simulink model "Parallel_RLC"  (R2025b)
settings: Solver=VariableStepAuto  StartTime=0.0  StopTime=0.03  RelTol=1e-7
libraries: fl_lib x8, nesl_utility x4, ee_lib x1
settings Model: Creator=franc  LastModifiedBy=franc

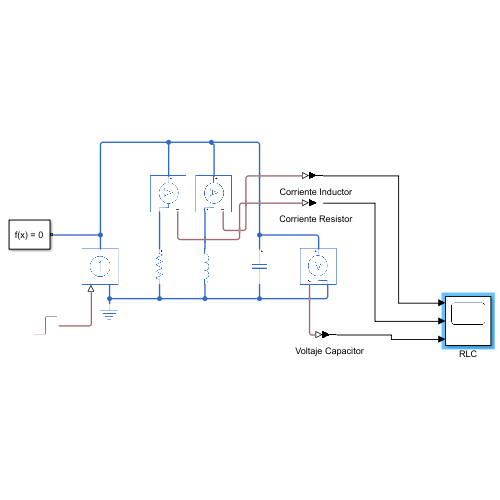
[thumbnail: Simulink's stored preview of the top-level diagram]
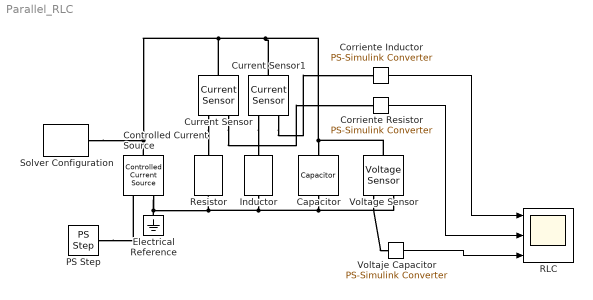
== system Parallel_RLC ==
  Capacitor : fl_lib/Electrical/Electrical Elements/Capacitor  c=2.53e-3 F  r=1e-6 Ohm  g=0 1/Ohm  i_specify=off  i_priority=None  i=0 A  i_nominal_specify=off  i_nominal_value=1  i_nominal_unit=A  v_specify=off  v_priority=None  v=0 V  v_nominal_specify=off  v_nominal_value=1  v_nominal_unit=V  vc_specify=off  vc_priority=High  vc=0 V  vc_nominal_specify=off  vc_nominal_value=1  vc_nominal_unit=V
  Controlled Current Source : fl_lib/Electrical/Electrical Sources/Controlled Current Source
  Corriente Inductor : nesl_utility/PS-Simulink Converter  PhysicalDomain=network_engine_domain  SubClassName=ps_output  LeftPortType=input  RightPortType=output  PseudoPeriodic=off  Frequencies=[]  VectorFormat=inherit  Unit=inherit  AffineConversion=off
  Corriente Resistor : nesl_utility/PS-Simulink Converter  PhysicalDomain=network_engine_domain  SubClassName=ps_output  LeftPortType=input  RightPortType=output  PseudoPeriodic=off  Frequencies=[]  VectorFormat=inherit  Unit=inherit  AffineConversion=off
  Current Sensor : fl_lib/Electrical/Electrical Sensors/Current Sensor
  Current Sensor1 : fl_lib/Electrical/Electrical Sensors/Current Sensor
  Electrical Reference : fl_lib/Electrical/Electrical Elements/Electrical Reference
  Inductor : ee_lib/Passive/Inductor  l=1e-3 H  enable_L_tol=ee.enum.toleranceApplication.none  L_tol=20  tol_distribution=ee.enum.toleranceDistribution.uniform  nSigma=4  r=0 Ohm  g=1e-9 1/Ohm  enable_operating_limits=ee.enum.enable.no  operating_limit_action=ee.enum.passive.reportOpLim.warn  max_working_current=1 A  power_rating=1 W  i_L_specify=off  i_L_priority=High  i_L=0 A  i_L_nominal_specify=off  i_L_nominal_value=1  i_L_nominal_unit=A
  PS Step : fl_lib/Physical Signals/Sources/PS Step  step_time=0 s  initial_value=0  final_value=1
  RLC : Scope  NumInputPorts=3
      settings: ActiveDisplayYMinimum=-0.16367566523078125  ActiveDisplayYMaximum=1.1801477523851314
  Resistor : fl_lib/Electrical/Electrical Elements/Resistor  R=0.449 Ohm  i_specify=off  i_priority=None  i=0 A  i_nominal_specify=off  i_nominal_value=1  i_nominal_unit=A  v_specify=off  v_priority=None  v=0 V  v_nominal_specify=off  v_nominal_value=1  v_nominal_unit=V
  Solver Configuration : nesl_utility/Solver Configuration  PhysicalDomain=network_engine_domain  SubClassName=solver  LeftPortType=input  RightPortType=generic  Tones=[]  Harmonics=[]  SimulateNoise=off  Profile=off  UseLocalSampling=off  EnableSwitchedLinearOptims=on  FrequencyDomain=off  UseCCode=off  RelTol=0.001  AbsTol=0.001  MinStep=1e-09  ToWorkspace=off  RevertToSquareIcSolve=off  NumHomotopyIterations=100  PhasorMode=off  PhasorModeNumHarmonics=1  ConsistencySolver=NEWTON_XTOL_AFTER_FTOL  IndexReductionMethod=DerivativeReplacement  DoDC=off  ResidualTolerance=1e-09  ConsistencyTolSource=GLOBAL  ConsistencyAbsTol=0.001  ConsistencyRelTol=0.001  ConsistencyTolFactor=0.5  UseLocalSolver=off  LocalSolverChoice=NE_BACKWARD_EULER_ADVANCER  ResolveIndetEquations=on  FunctionEvalNumThread=1  LocalSolverSampleTime=0.001  DoFixedCost=off  MaxNonlinIter=3  MaxModeIter=2  ComputeImpulses=off  ImpulseIterations=2  LinearAlgebra=auto  LinearAlgebraNumThread=0  EquationFormulation=NE_TIME_EF  DelaysMemoryBudget=1024  AutomaticFiltering=on  FilteringTimeConstant=0.001  PartitionStorageMethod=AS_NEEDED  PartitionMemoryBudget=1024  PartitionMethod=ROBUST  MultibodyUseLocalSolver=off  MultibodyLocalSolverChoice=ODE1  MultibodyLocalSolverSampleTime=0.001
  Voltage Sensor : fl_lib/Electrical/Electrical Sensors/Voltage Sensor
  Voltaje Capacitor : nesl_utility/PS-Simulink Converter  PhysicalDomain=network_engine_domain  SubClassName=ps_output  LeftPortType=input  RightPortType=output  PseudoPeriodic=off  Frequencies=[]  VectorFormat=inherit  Unit=inherit  AffineConversion=off
  wires:
  Voltaje Capacitor/1 -> RLC/3
  Corriente Inductor/1 -> RLC/1
  Corriente Resistor/1 -> RLC/2
  connections:
  Controlled Current Source/LConn1 -- Solver Configuration/RConn1 -- Current Sensor1/LConn1 -- Voltage Sensor/LConn1 -- Capacitor/LConn1 -- Current Sensor/LConn1
  Controlled Current Source/RConn2 -- Electrical Reference/LConn1 -- Voltage Sensor/RConn2 -- Capacitor/RConn1 -- Inductor/RConn1 -- Resistor/RConn1
  PS Step/RConn1 -- Controlled Current Source/RConn1
  Voltage Sensor/RConn1 -- Voltaje Capacitor/LConn1
  Current Sensor/RConn2 -- Resistor/LConn1
  Current Sensor1/RConn2 -- Inductor/LConn1
  Current Sensor1/RConn1 -- Corriente Inductor/LConn1
  Current Sensor/RConn1 -- Corriente Resistor/LConn1
